simulink model "turbo_controller"  (R2025a)
settings: Solver=FixedStepAuto  StartTime=0.0  StopTime=inf  FixedStep=0.001  RelTol=1e-3
PostLoadFcn:
  | % 自动定位同目录CubeMX文件；不需要外部初始化脚本。
  | codertarget.data.setParameterValue('turbo_controller','STM32CubeMX.ProjectFile',fullfile(fileparts(get_param('turbo_controller','FileName')),'turbo_f407.ioc'));
InitFcn:
  | % 中文说明：按原控制器字段与类型创建三组接口总线；控制参数已内嵌。
  | tc_names=["EValve_Cycle" "EValve_Open" "Eblast_Cycle" "Eblast_Open" "Motor_Cycle" "Motor_Open" "EValve_Enable" "Eblast_Enable" "Motor_Enable" "SWO_Firework" "SWO_BleedAir" "EngineState" "Flag_ECUReset_Clear" "Flag_ECUReset_Save" "Flag_Reset_Enable" "Accelerator" "Nc_dem" "Nc"]; tc_types=["uint16" "uint16" "uint16" "uint16" "uint16" "uint16" "uint8" "uint8" "uint8" "uint8" "uint8" "uint8" "uint8" "uint8" "uint8" "single" "single" "single"];
  | for tc_k=1:numel(tc_names)
  |  tc_e(tc_k)=Simulink.BusElement; tc_e(tc_k).Name=char(tc_names(tc_k)); tc_e(tc_k).DataType=char(tc_types(tc_k));
  | end
  | EngineControl_Out=Simulink.Bus; EngineControl_Out.DataScope='Exported'; EngineControl_Out.Elements=tc_e;
  | clear tc_e tc_names tc_types tc_k
  | tc_names=["savedata1" "savedata2" "savedata3" "savedata4" "savedata5" "savedata6" "savedata7" "savedata8" "savedata9" "savedata10" "savedata11" "savedata12" "savedata13" "savedata14" "savedata15" "savedata16" "savedata17" "savedata18" "savedata19" "savedata20" "savedata21" "savedata22" "savedata23" "savedata24" "savedata25"]; tc_types=["single" "single" "single" "single" "single" "single" "single" "single" "single" "single" "single" "single" "single" "single" "single" "single" "single" "single" "single" "single" "single" "single" "single" "single" "single"];
  | for tc_k=1:numel(tc_names)
  |  tc_e(tc_k)=Simulink.BusElement; tc_e(tc_k).Name=char(tc_names(tc_k)); tc_e(tc_k).DataType=char(tc_types(tc_k));
  | end
  | SaveData_Out=Simulink.Bus; SaveData_Out.DataScope='Exported'; SaveData_Out.Elements=tc_e;
  | clear tc_e tc_names tc_types tc_k
  | tc_names=["senddata1" "senddata2" "senddata3" "senddata4" "senddata5" "senddata6" "senddata7" "senddata8" "senddata9" "senddata10" "senddata11" "senddata12" "senddata13" "senddata14" "senddata15" "senddata16" "senddata17" "senddata18" "senddata19" "senddata20" "senddata21" "senddata22" "senddata23" "senddata24" "senddata25" "senddata26" "senddata27" "senddata28" "senddata29"]; tc_types=["uint8" "uint8" "uint8" "uint8" "uint8" "uint8" "uint8" "uint8" "uint8" "uint8" "uint8" "uint8" "uint8" "uint8" "uint8" "uint8" "uint8" "uint8" "uint8" "uint8" "uint8" "uint8" "uint8" "uint8" "uint8" "uint8" "uint8" "uint8" "uint8"];
  | for tc_k=1:numel(tc_names)
  |  tc_e(tc_k)=Simulink.BusElement; tc_e(tc_k).Name=char(tc_names(tc_k)); tc_e(tc_k).DataType=char(tc_types(tc_k));
  | end
  | SendData_Out=Simulink.Bus; SendData_Out.DataScope='Exported'; SendData_Out.Elements=tc_e;
  | clear tc_e tc_names tc_types tc_k
  | 
  | % 以下为接口中文说明；只设置描述，不改变数值或数据类型。
  | EngineControl_Out.Description='执行控制输出（阀、电机、点火、状态及复位请求）';
  | tc_cn=["EValve_Cycle（主油阀周期计数（每计数2毫秒））" "EValve_Open（主油阀开通计数（每计数2毫秒））" "Eblast_Cycle（副油阀周期计数（每计数2毫秒））" "Eblast_Open（副油阀开通计数（每计数2毫秒））" "Motor_Cycle（起动电机周期计数）" "Motor_Open（起动电机开通计数）" "EValve_Enable（主油阀驱动使能）" "Eblast_Enable（副油阀驱动使能）" "Motor_Enable（起动电机使能）" "SWO_Firework（点火器使能（1开））" "SWO_BleedAir（引气阀使能（1开））" "EngineState（发动机状态）" "Flag_ECUReset_Clear（清除复位恢复状态请求）" "Flag_ECUReset_Save（保存复位恢复数据请求）" "Flag_Reset_Enable（处理器软件复位请求）" "Accelerator（油门／油泵给定控制量）" "Nc_dem（控制目标转速）" "Nc（发动机反馈转速（转每分））"];
  | tc_elements=EngineControl_Out.Elements;
  | for tc_k=1:numel(tc_cn)
  |  tc_elements(tc_k).Description=char(tc_cn(tc_k));
  | end
  | EngineControl_Out.Elements=tc_elements;
  | clear tc_cn tc_elements tc_k
  | SaveData_Out.Description='25项运行记录；字段含义按当前模型数据来源解释';
  | tc_cn=["savedata1（指令回显记录）" "savedata2（入口总温记录（℃））" "savedata3（电源电压记录）" "savedata4（排气温度记录（℃））" "savedata5（标定燃油压力记录）" "savedata6（副油阀占空比记录（％））" "savedata7（主油阀占空比记录（％））" "savedata8（温度修正转速记录）" "savedata9（开关输出及反馈位域）" "savedata10（物理转速记录）" "savedata11（油泵目标给定原始值）" "savedata12（起动电机占空比记录（％））" "savedata13（发动机状态码记录）" "savedata14（故障告警位域记录）" "savedata15（模型记录帧序号）" "savedata16（处理器温度记录（℃））" "savedata17（装订转速记录（沿用旧电源字段名））" "savedata18（导航高度记录）" "savedata19（飞行空速记录）" "savedata20（主阀旧记录位（恒零保留））" "savedata21（第21项保留记录（恒零））" "savedata22（保留记录项22）" "savedata23（保留记录项23）" "savedata24（保留记录项24）" "savedata25（保留记录项25）"];
  | tc_elements=SaveData_Out.Elements;
  | for tc_k=1:numel(tc_cn)
  |  tc_elements(tc_k).Description=char(tc_cn(tc_k));
  | end
  | SaveData_Out.Elements=tc_elements;
  | clear tc_cn tc_elements tc_k
  | SendData_Out.Description='29字段回传及外设命令接口；板端上位机帧只取第3至27字段';
  | tc_cn=["senddata1（回传发送允许标志（不直接上线路））" "senddata2（回传载荷长度25字节）" "senddata3（回传指令回显字节）" "senddata4（总温编码字节（℃＋80））" "senddata5（电源电压编码字节）" "senddata6（排温编码高字节）" "senddata7（排温编码低字节）" "senddata8（燃油压力编码高字节）" "senddata9（燃油压力编码低字节）" "senddata10（副油阀占空比字节（％））" "senddata11（主油阀占空比字节（％））" "senddata12（修正转速编码高字节）" "senddata13（修正转速编码低字节）" "senddata14（驱动及反馈状态位域）" "senddata15（物理转速编码高字节）" "senddata16（物理转速编码低字节）" "senddata17（油泵目标给定高字节（串口二使用））" "senddata18（油泵目标给定低字节（串口二使用））" "senddata19（起动电机占空比命令（串口一使用））" "senddata20（发动机状态码字节）" "senddata21（故障告警位域字节）" "senddata22（帧序号占位（板端另行填写））" "senddata23（处理器温度编码（℃＋50））" "senddata24（控制目标转速编码高字节）" "senddata25（控制目标转速编码低字节）" "senddata26（占位字节（板端改填实测泵速高字节））" "senddata27（占位字节（板端改填实测泵速低字节））" "senddata28（装订转速高字节（本板未发送））" "senddata29（装订转速低字节（本板未发送））"];
  | tc_elements=SendData_Out.Elements;
  | for tc_k=1:numel(tc_cn)
  |  tc_elements(tc_k).Description=char(tc_cn(tc_k));
  | end
  | SendData_Out.Elements=tc_elements;
  | clear tc_cn tc_elements tc_k
  | 
  | 
  | % FRAM模块化事务：接口类型和上电初始状态，随模型保存，无外部初始化文件。
  | clear FM_elements
  | FM_elements(1)=Simulink.BusElement;FM_elements(1).Name='phase';FM_elements(1).DataType='uint8';FM_elements(1).Dimensions=[1 1];FM_elements(1).Description='phase（当前事务阶段）';
  | FM_elements(2)=Simulink.BusElement;FM_elements(2).Name='a';FM_elements(2).DataType='uint8';FM_elements(2).Dimensions=[64 1];FM_elements(2).Description='a（启动时缓存的首区64字节）';
  | FM_elements(3)=Simulink.BusElement;FM_elements(3).Name='active';FM_elements(3).DataType='uint16';FM_elements(3).Dimensions=[1 1];FM_elements(3).Description='active（当前有效记录区地址）';
  | FM_elements(4)=Simulink.BusElement;FM_elements(4).Name='generation';FM_elements(4).DataType='uint32';FM_elements(4).Dimensions=[1 1];FM_elements(4).Description='generation（当前有效记录代号）';
  | FM_elements(5)=Simulink.BusElement;FM_elements(5).Name='record';FM_elements(5).DataType='uint8';FM_elements(5).Dimensions=[64 1];FM_elements(5).Description='record（本次冻结的待写记录）';
  | FM_elements(6)=Simulink.BusElement;FM_elements(6).Name='addr';FM_elements(6).DataType='uint16';FM_elements(6).Dimensions=[1 1];FM_elements(6).Description='addr（本次备用写入地址）';
  | FM_elements(7)=Simulink.BusElement;FM_elements(7).Name='lastSave';FM_elements(7).DataType='single';FM_elements(7).Dimensions=[1 1];FM_elements(7).Description='lastSave（上次开始保存的秒数）';
  | FM_elements(8)=Simulink.BusElement;FM_elements(8).Name='lastState';FM_elements(8).DataType='uint8';FM_elements(8).Dimensions=[1 1];FM_elements(8).Description='lastState（上次保存时的发动机状态）';
  | FM_elements(9)=Simulink.BusElement;FM_elements(9).Name='boot';FM_elements(9).DataType='boolean';FM_elements(9).Dimensions=[1 1];FM_elements(9).Description='boot（启动记录是否允许恢复）';
  | FM_elements(10)=Simulink.BusElement;FM_elements(10).Name='consumed';FM_elements(10).DataType='boolean';FM_elements(10).Dimensions=[1 1];FM_elements(10).Description='consumed（本次启动恢复通知是否已发送）';
  | FM_elements(11)=Simulink.BusElement;FM_elements(11).Name='payload';FM_elements(11).DataType='uint8';FM_elements(11).Dimensions=[20 1];FM_elements(11).Description='payload（当前20字节恢复内容）';
  | ... (+35 lines)
model workspace (MAT data in the model file):
  CRC16_Table_Reference = [0 4129 8258 12387 16516 20645 24774 28903 33032 37161 41290 45419 ... (256 elements, 256x1)]
  PE_Kaer = [0.15402 0.15402 0.12264 0.10076 0.09481 0.07601 0.07111 0.0569 0.05198 0.04926 0.05308 0.04325 ... (13 elements, 1x13)]
  PE_Nr = [21.2982 61.4260372 67.7475458 72.7394382 76.845934 80.6988798 83.8449282 86.6491912 88.9382406 89.178606 91.1938214 93.4068058 ... (13 elements, 1x13)]
  PE_Pump_Translate = 33.5999984741
  PE_RotaSpeed_Translate = 860
  PE_Taer = [0.4939154 0.4939154 0.40780982 0.34066978 0.31622756 0.30405716 0.34300244 0.26785022 0.37393554 0.23914836 0.44563948 0.31044662 ... (13 elements, 1x13)]
  PF_ACCFULLRANGE = 3360
  PF_Flag_ECUReset = 0
  PF_Flag_rx_suc = 1
  PF_Gear_Info = [40000; 45000; 50000; 55000; 57000; 59000; 60000; 61000; 61000; 61000; 61000; 61000]
  PF_K_TiaoJie = 1
  PF_Kpu = 10
  PF_MySet_Rxdata = [0 0 0 0 0 0 0 0 0 0 0 0 ... (50 elements, 50x1)]
  PF_MyUsart1_Rxdata = [0 0 0 0 0 0 0 0 0 0 0 0 ... (50 elements, 50x1)]
  PF_MyUsart2_Rxdata = [0 0 0 0 0 0 0 0 0 0 0 0 ... (50 elements, 50x1)]
  PF_Reset_Information = [0 0 0 0 0 0 0 0 0 0 0 0 ... (20 elements, 20x1)]
  PF_Sensor_X1_T4 = [0 4095]
  PF_Sensor_X2_T4 = [0 1.66666698456]
  PF_Sensor_X3_T4 = [0 504 999 1497 2010 2529 3051 3568 4076 4571 4959]
  PF_Sensor_X_P2 = [0.5 3]
  PF_Sensor_X_Poil = [0.5 3]
  PF_Sensor_X_T1t = [-50 300]
  PF_Sensor_X_Vpower = [0 3]
  PF_Sensor_X_Vpump = [0 3]
  PF_Sensor_Y1_T4 = [0 3]
  PF_Sensor_Y2_T4 = [0 5000]
  PF_Sensor_Y3_T4 = [0 100 200 300 400 500 600 700 800 900 980]
  PF_Sensor_Y_P2 = [0 1000]
  PF_Sensor_Y_Poil = [0 1000]
  PF_Sensor_Y_T1t = [-50 300]
  PF_Sensor_Y_Vpower = [0 33]
  PF_Sensor_Y_Vpump = [0 33]
  PG_CtrlMode_CloseLoop : mpt.Parameter (value not decoded)
  PG_CtrlMode_ManualAcc : mpt.Parameter (value not decoded)
  PG_CtrlMode_Origin : mpt.Parameter (value not decoded)
  PG_CtrlMode_Start : mpt.Parameter (value not decoded)
  PG_CtrlMode_Stop : mpt.Parameter (value not decoded)
  PG_ES_Clp : mpt.Parameter (value not decoded)
  PG_ES_EngStart : mpt.Parameter (value not decoded)
  PG_ES_Manual : mpt.Parameter (value not decoded)
  PG_ES_Origin : mpt.Parameter (value not decoded)
  PG_ES_Stop : mpt.Parameter (value not decoded)
  PG_Instr_BleedAirSet : mpt.Parameter (value not decoded)
  PG_Instr_CloseLoop : mpt.Parameter (value not decoded)
  PG_Instr_ECUReSet : mpt.Parameter (value not decoded)
  PG_Instr_EValveSet : mpt.Parameter (value not decoded)
  PG_Instr_EblastSet : mpt.Parameter (value not decoded)
  PG_Instr_Erase : mpt.Parameter (value not decoded)
  PG_Instr_FireWorkSet : mpt.Parameter (value not decoded)
  PG_Instr_ManualPlus : mpt.Parameter (value not decoded)
  PG_Instr_ManualrReduce : mpt.Parameter (value not decoded)
  PG_Instr_MotorSet : mpt.Parameter (value not decoded)
  PG_Instr_OilSet : mpt.Parameter (value not decoded)
  PG_Instr_SelfCheck : mpt.Parameter (value not decoded)
  PG_Instr_Start : mpt.Parameter (value not decoded)
  PG_Instr_Stop : mpt.Parameter (value not decoded)
  PG_Instr_StopZero : Simulink.Parameter (value not decoded)
  PG_Location_Air : Simulink.Parameter (value not decoded)
  PG_Location_Gnd : Simulink.Parameter (value not decoded)
  PG_ServoCtrlMode_CloseLoop : Simulink.Parameter (value not decoded)
  PG_ServoCtrlMode_CloseLoopMax : Simulink.Parameter (value not decoded)
  PG_ServoCtrlMode_CloseLoopMin : Simulink.Parameter (value not decoded)
  PG_ServoCtrlMode_ManualAcc : Simulink.Parameter (value not decoded)
  PG_ServoCtrlMode_ManualAccMax : Simulink.Parameter (value not decoded)
  PG_ServoCtrlMode_ManualAccMin : Simulink.Parameter (value not decoded)
  PG_SpeedDot_Permit : Simulink.Parameter (value not decoded)
  PL_EngineModel_Actuator = [0 10 100]
  PL_EngineModel_EngineStar_Press_P2 = [1013 1098.4 1099.144828 1099.931034 1103.613793 1162.662069 1143.793103 1131.006897 1123.186207 1117.6 1114 1111.806897 ... (127 elements, 1x127)]
  PL_EngineModel_EngineStar_RotaSpeed = [200 2000 9584 9660 10220 10240 10260 10288 10308 10368 10380 10408 ... (127 elements, 1x127)]
  PL_EngineModel_EngineStar_Temp_Exhaust = [128 129 129.1 130 131 131.1 132 133 134 134.1 135 135.1 ... (127 elements, 1x127)]
  PL_EngineModel_EngineStar_Time = [0.05 0.1 0.15 0.2 0.25 0.3 0.35 0.4 0.45 0.5 0.55 0.6 ... (127 elements, 1x127)]
  PL_EngineModel_IdleAbove_Nr = [0 21.2982 61.4260372 67.7475458 72.7394382 76.845934 80.6988798 83.8449282 86.6491912 88.9382406 89.178606 91.1938214 ... (14 elements, 1x14)]
  PL_EngineModel_IdleAbove_P2r = [0.986923266716 1.57907722675 1.81593881076 1.99358499877 2.23044658278 2.43770046879 2.65482358747 2.84233900814 3.03972366149 3.18776215149 3.25684678016 3.3950160375 ... (14 elements, 1x14)]
  PL_EngineModel_IdleAbove_Tempr = [0.0536001429337 1.07200285867 1.63301768805 1.63659103091 1.66875111667 1.72592460247 1.77595140254 1.86171163123 1.95461854565 2.03323208862 2.03323208862 2.13685903162 ... (14 elements, 1x14)]
  PL_EngineModel_IdleAbove_Ter = [0.42434128 0.42434128 0.42434128 0.30669408 0.23570008 0.22150128 0.1997974 0.23803274 0.16115638 0.24279948 0.13600422 0.31308354 ... (14 elements, 1x14)]
  PL_EngineModel_IdleAbove_Wfr = [0 10.142 23.8337 27.8905 31.9473 36.0041 40.0609 44.1177 48.1745 52.2313 52.7384 56.7952 ... (14 elements, 1x14)]
  PL_EngineModel_Press_P2 = [400 400 400 400 400 400 400 400 400 400]
  PL_EngineModel_Rotaspeed = [0 20000 96400]
  PL_EngineModel_Temp_Exhaust = [500 500 500 500 500 500 500 500 500 500]
  PL_Kaer = [0.1 0.1 0.1 0.1 0.1 0.1]
  PL_Nr = [50 60 70 80 90 100]
  PL_Taer = [0.1 0.1 0.1 0.1 0.1 0.1]
  Sig : Simulink.Signal (value not decoded)
  Ts_ms : Simulink.Parameter (value not decoded)
  false : Simulink.Parameter (value not decoded)
  true : Simulink.Parameter (value not decoded)
symbols that are objects in the model workspace (value not decoded): PG_CtrlMode_CloseLoop, PG_CtrlMode_ManualAcc, PG_CtrlMode_Origin, PG_CtrlMode_Start, PG_CtrlMode_Stop, PG_ES_Clp, PG_ES_EngStart, PG_ES_Manual, PG_ES_Origin, PG_ES_Stop, PG_Instr_BleedAirSet, PG_Instr_CloseLoop, PG_Instr_EblastSet, PG_Instr_ECUReSet, PG_Instr_Erase, PG_Instr_EValveSet, PG_Instr_FireWorkSet, PG_Instr_ManualPlus, PG_Instr_ManualrReduce, PG_Instr_MotorSet, PG_Instr_OilSet, PG_Instr_SelfCheck, PG_Instr_Start, PG_Instr_Stop, PG_Instr_StopZero, PG_ServoCtrlMode_CloseLoop, PG_ServoCtrlMode_CloseLoopMax, PG_ServoCtrlMode_CloseLoopMin, PG_ServoCtrlMode_ManualAcc, PG_ServoCtrlMode_ManualAccMax, PG_ServoCtrlMode_ManualAccMin, Ts_ms
libraries: simulink x97, stm32blockslib x10, stm32f4xxblockslib x8
(part 24 of 26)

== system turbo_controller/BoardInput_输入换算与协议解析/In03_Pump（油泵回包预留校验）/Receive（逐字节组帧与保持有效结果）_353/Step03_收齐且校验通过才接受/Verify（完整帧校验）_344/CRC16（循环冗余校验）_328/TableStep（查表更新本字节校验） ==
  note: CRC16的一个字节怎样查表更新
      |
      | 父级已经把当前数据字节异或进旧CRC的高8位，形成Merged。本模块把这个16位数拆成“用哪项表”和
      | “保留哪些移位结果”两部分。
      |
      | 先取高8位：索引=floor(Merged/256)，范围0～255。用它到CRC16_Table_Reference查表；模型Select
      | or按零基索引取值，写成MATLAB数组下标时要用索引+1。
      | 另一条支路把Merged左移一个字节，即乘256，然后只保留低16位：移位值=bitand(uint32(Merged)×25
      | 6,65535)。
      |
      | 最后将表值与移位值按位异或：
      | 新CRC=bitxor(表值,移位值)。
      |
      | 例如Merged=十六进制1234，高8位12用于选表项，左移并截16位后为3400，再与表项异或。宽类型uint
      | 32是为了中间计算不先溢出，并不表示输出CRC变成32位。结果回到父级，继续处理下一个数据字节。
  note: 【中文学习说明：一次查表更新一个字节】
      | 一、输入已经是“旧CRC XOR (当前字节×256)”。
      | 输入是16位无符号整数，记作Merged（合并值）。
      |
      | 二、上路得到查表下标。
      | 合并值÷256后向下取整，取得高八位，范围0～255。
      | 这等价于参考程序中的“旧CRC高字节 XOR 当前字节”。
      | Lookup（按下标取表项）采用Zero-based（从0编号），
      | 所以0就取表的第一项，255取最后一项，不能再加1。
      |
      | 三、下路准备左移结果。
      | 先转uint32（32位无符号数），再乘256左移8位，
      | 与65535作按位AND，只保留低16位，最后转回uint16。
      | 先加宽再移位，是为了避免整数饱和破坏结果。
      | 当前字节已经在高8位，左移后移出16位范围，
      | 因此截断后与“旧CRC左移8位”的结果相同。
      |
      | 四、两路按位XOR（异或），输出更新后的16位CRC。
      | 异或的意思：两个二进制位相同得0，不同得1。
      | 本页不需要循环和记忆，输入一到就能按组合逻辑计算；
      | 跨字节的累计和每帧初值由父级CRC16模块负责。
      |
      | 五、CRC16Table（查表数据）是256项整数常量。
      | 表内容逐项复制自参考工程USER/crc.c，
      | 与NRIST_lib/NRIST_calculate.c中的表一致。
      | Selector（按下标选取）直接取一项，不做曲线插值。
      | 表中数值不是需要现场调节的控制参数。
  Merged（旧校验值与当前字节异或后的数） : Inport  OutDataTypeStr=uint16
  CRC16Table（参考工程原始二百五十六项表） : Constant  Value=CRC16_Table_Reference  OutDataTypeStr=uint16
  Divisor（高字节换算除数） : Constant  Value=256  OutDataTypeStr=double
  Exact（转双精度做精确除法） : DataTypeConversion  OutDataTypeStr=double  SaturateOnIntegerOverflow=off  RndMeth=Floor
  HighByte（除二百五十六取高字节） : Product  Inputs=*/  OutDataTypeStr=double
  Index（向下取整得到零至二百五十五） : DataTypeConversion  OutDataTypeStr=uint32  RndMeth=Floor
  LeftByte（左移一个字节） : Product  Inputs=**  OutDataTypeStr=uint32  SaturateOnIntegerOverflow=on
  Lookup（按零基索引读取校验表） : Selector  IndexMode=Zero-based  InputPortWidth=256  IndexOptions=Index vector (port)  Indices=1  OutputSizes=1
  Mask16（保留低十六位） : Constant  Value=65535  OutDataTypeStr=uint32
  Shift16（移位结果转十六位） : DataTypeConversion  OutDataTypeStr=uint16  SaturateOnIntegerOverflow=off  RndMeth=Floor
  ShiftBase（一个字节的移位系数） : Constant  Value=256  OutDataTypeStr=uint32
  Update（查表值与移位结果异或） : simulink/Logic and Bit Operations/Bitwise Operator  logicop=XOR  UseBitMask=off  NumInputPorts=2  BitMask=bin2dec('11011001')  BitMaskRealWorld=Stored Integer
      settings: LibrarySourceBlock=|
      | hdlsllib/Logic and Bit
      | Operations/Bitwise
      | Operator
  Wide（转三十二位防止移位溢出） : DataTypeConversion  OutDataTypeStr=uint32  SaturateOnIntegerOverflow=off  RndMeth=Floor
  Wrap16（截取左移后的低十六位） : simulink/Logic and Bit Operations/Bitwise Operator  logicop=AND  UseBitMask=off  NumInputPorts=2  BitMask=bin2dec('11011001')  BitMaskRealWorld=Stored Integer
      settings: LibrarySourceBlock=|
      | hdlsllib/Logic and Bit
      | Operations/Bitwise
      | Operator
  CRC（本字节处理后的校验值） : Outport
  wires:
  Merged（旧校验值与当前字节异或后的数）/1 -> Wide（转三十二位防止移位溢出）/1, Exact（转双精度做精确除法）/1
  Wide（转三十二位防止移位溢出）/1 -> LeftByte（左移一个字节）/1
  ShiftBase（一个字节的移位系数）/1 -> LeftByte（左移一个字节）/2
  LeftByte（左移一个字节）/1 -> Wrap16（截取左移后的低十六位）/1
  Mask16（保留低十六位）/1 -> Wrap16（截取左移后的低十六位）/2
  Wrap16（截取左移后的低十六位）/1 -> Shift16（移位结果转十六位）/1
  Exact（转双精度做精确除法）/1 -> HighByte（除二百五十六取高字节）/1
  Divisor（高字节换算除数）/1 -> HighByte（除二百五十六取高字节）/2
  HighByte（除二百五十六取高字节）/1 -> Index（向下取整得到零至二百五十五）/1
  CRC16Table（参考工程原始二百五十六项表）/1 -> Lookup（按零基索引读取校验表）/1
  Index（向下取整得到零至二百五十五）/1 -> Lookup（按零基索引读取校验表）/2
  Lookup（按零基索引读取校验表）/1 -> Update（查表值与移位结果异或）/1
  Shift16（移位结果转十六位）/1 -> Update（查表值与移位结果异或）/2
  Update（查表值与移位结果异或）/1 -> CRC（本字节处理后的校验值）/1

== system turbo_controller/BoardOutput_串口封装与阀门时序/Out01_Pump（泵反馈解析与滤波）/Receive（逐字节组帧与保持有效结果）_680/Step03_收齐且校验通过才接受/Verify（完整帧校验）_662/CRC16（循环冗余校验）_646/TableStep（查表更新本字节校验） ==
  note: CRC16的一个字节怎样查表更新
      |
      | 父级已经把当前数据字节异或进旧CRC的高8位，形成Merged。本模块把这个16位数拆成“用哪项表”和
      | “保留哪些移位结果”两部分。
      |
      | 先取高8位：索引=floor(Merged/256)，范围0～255。用它到CRC16_Table_Reference查表；模型Select
      | or按零基索引取值，写成MATLAB数组下标时要用索引+1。
      | 另一条支路把Merged左移一个字节，即乘256，然后只保留低16位：移位值=bitand(uint32(Merged)×25
      | 6,65535)。
      |
      | 最后将表值与移位值按位异或：
      | 新CRC=bitxor(表值,移位值)。
      |
      | 例如Merged=十六进制1234，高8位12用于选表项，左移并截16位后为3400，再与表项异或。宽类型uint
      | 32是为了中间计算不先溢出，并不表示输出CRC变成32位。结果回到父级，继续处理下一个数据字节。
  note: 【中文学习说明：一次查表更新一个字节】
      | 一、输入已经是“旧CRC XOR (当前字节×256)”。
      | 输入是16位无符号整数，记作Merged（合并值）。
      |
      | 二、上路得到查表下标。
      | 合并值÷256后向下取整，取得高八位，范围0～255。
      | 这等价于参考程序中的“旧CRC高字节 XOR 当前字节”。
      | Lookup（按下标取表项）采用Zero-based（从0编号），
      | 所以0就取表的第一项，255取最后一项，不能再加1。
      |
      | 三、下路准备左移结果。
      | 先转uint32（32位无符号数），再乘256左移8位，
      | 与65535作按位AND，只保留低16位，最后转回uint16。
      | 先加宽再移位，是为了避免整数饱和破坏结果。
      | 当前字节已经在高8位，左移后移出16位范围，
      | 因此截断后与“旧CRC左移8位”的结果相同。
      |
      | 四、两路按位XOR（异或），输出更新后的16位CRC。
      | 异或的意思：两个二进制位相同得0，不同得1。
      | 本页不需要循环和记忆，输入一到就能按组合逻辑计算；
      | 跨字节的累计和每帧初值由父级CRC16模块负责。
      |
      | 五、CRC16Table（查表数据）是256项整数常量。
      | 表内容逐项复制自参考工程USER/crc.c，
      | 与NRIST_lib/NRIST_calculate.c中的表一致。
      | Selector（按下标选取）直接取一项，不做曲线插值。
      | 表中数值不是需要现场调节的控制参数。
  Merged（旧校验值与当前字节异或后的数） : Inport  OutDataTypeStr=uint16
  CRC16Table（参考工程原始二百五十六项表） : Constant  Value=CRC16_Table_Reference  OutDataTypeStr=uint16
  Divisor（高字节换算除数） : Constant  Value=256  OutDataTypeStr=double
  Exact（转双精度做精确除法） : DataTypeConversion  OutDataTypeStr=double  SaturateOnIntegerOverflow=off  RndMeth=Floor
  HighByte（除二百五十六取高字节） : Product  Inputs=*/  OutDataTypeStr=double
  Index（向下取整得到零至二百五十五） : DataTypeConversion  OutDataTypeStr=uint32  RndMeth=Floor
  LeftByte（左移一个字节） : Product  Inputs=**  OutDataTypeStr=uint32  SaturateOnIntegerOverflow=on
  Lookup（按零基索引读取校验表） : Selector  IndexMode=Zero-based  InputPortWidth=256  IndexOptions=Index vector (port)  Indices=1  OutputSizes=1
  Mask16（保留低十六位） : Constant  Value=65535  OutDataTypeStr=uint32
  Shift16（移位结果转十六位） : DataTypeConversion  OutDataTypeStr=uint16  SaturateOnIntegerOverflow=off  RndMeth=Floor
  ShiftBase（一个字节的移位系数） : Constant  Value=256  OutDataTypeStr=uint32
  Update（查表值与移位结果异或） : simulink/Logic and Bit Operations/Bitwise Operator  logicop=XOR  UseBitMask=off  NumInputPorts=2  BitMask=bin2dec('11011001')  BitMaskRealWorld=Stored Integer
      settings: LibrarySourceBlock=|
      | hdlsllib/Logic and Bit
      | Operations/Bitwise
      | Operator
  Wide（转三十二位防止移位溢出） : DataTypeConversion  OutDataTypeStr=uint32  SaturateOnIntegerOverflow=off  RndMeth=Floor
  Wrap16（截取左移后的低十六位） : simulink/Logic and Bit Operations/Bitwise Operator  logicop=AND  UseBitMask=off  NumInputPorts=2  BitMask=bin2dec('11011001')  BitMaskRealWorld=Stored Integer
      settings: LibrarySourceBlock=|
      | hdlsllib/Logic and Bit
      | Operations/Bitwise
      | Operator
  CRC（本字节处理后的校验值） : Outport
  wires:
  Merged（旧校验值与当前字节异或后的数）/1 -> Wide（转三十二位防止移位溢出）/1, Exact（转双精度做精确除法）/1
  Wide（转三十二位防止移位溢出）/1 -> LeftByte（左移一个字节）/1
  ShiftBase（一个字节的移位系数）/1 -> LeftByte（左移一个字节）/2
  LeftByte（左移一个字节）/1 -> Wrap16（截取左移后的低十六位）/1
  Mask16（保留低十六位）/1 -> Wrap16（截取左移后的低十六位）/2
  Wrap16（截取左移后的低十六位）/1 -> Shift16（移位结果转十六位）/1
  Exact（转双精度做精确除法）/1 -> HighByte（除二百五十六取高字节）/1
  Divisor（高字节换算除数）/1 -> HighByte（除二百五十六取高字节）/2
  HighByte（除二百五十六取高字节）/1 -> Index（向下取整得到零至二百五十五）/1
  CRC16Table（参考工程原始二百五十六项表）/1 -> Lookup（按零基索引读取校验表）/1
  Index（向下取整得到零至二百五十五）/1 -> Lookup（按零基索引读取校验表）/2
  Lookup（按零基索引读取校验表）/1 -> Update（查表值与移位结果异或）/1
  Shift16（移位结果转十六位）/1 -> Update（查表值与移位结果异或）/2
  Update（查表值与移位结果异或）/1 -> CRC（本字节处理后的校验值）/1

== stateflow chart turbo_controller/MAM/Timmer_ms1 ==
  note: 确认越限是否持续达到指定时间
      |
      | 输入越限条件成立时累计次数；不成立时按图内复位分支清除本次确认。到Time_ms/Ts_ms对应的门限
      | 后，输出持续越限标志。
      |
      | 父级给定约2000 ms，Ts_ms=20 ms，相当于约100次连续调用。温度或转速只超过一拍后恢复，不会累
      | 计成连续2 s。该定时只用于告警确认，不改变测量值，也不对排温或转速再次滤波。
  (default) -> (junction 26)
    settings: description=无附加条件的迁移路径，执行次序1；沿本图当前连接推进。
  (junction 26) -> (junction 3) [order 1] : [true/*真值*/ == In/*输入*/]
    settings: description=本路径的判据/动作：[true == In]。执行次序1；条件成立才执行本箭头动作。
  (junction 3) -> (junction 5) [order 1] : [Cnt/*计数器*/ >= uint32/*三十二位无符号整数*/(100000)]
    settings: description=本路径的判据/动作：[Cnt >= uint32(100000)]。执行次序1；条件成立才执行本箭头动作。
  (junction 26) -> (junction 43) [order 2] : {Cnt/*计数器*/ = 0;Out/*输出*/ = false/*假值*/;}
    settings: description=本路径的判据/动作：{Cnt = 0;Out = false;}。执行次序2；条件成立才执行本箭头动作。
  (junction 3) -> (junction 10) [order 2] : {Cnt/*计数器*/++;}
    settings: description=本路径的判据/动作：{Cnt++;}。执行次序2；条件成立才执行本箭头动作。
  (junction 5) -> (junction 12) : {Cnt/*计数器*/ = 100000;}
    settings: description=本路径的判据/动作：{Cnt = 100000;}。执行次序1；条件成立才执行本箭头动作。
  (junction 12) -> (junction 10)
    settings: description=无附加条件的迁移路径，执行次序1；沿本图当前连接推进。
  (junction 10) -> (junction 30)
    settings: description=无附加条件的迁移路径，执行次序1；沿本图当前连接推进。
  (junction 30) -> (junction 33) [order 1] : [Cnt/*计数器*/ >uint32/*三十二位无符号整数*/(Time_ms/*时间毫秒*//Ts_ms/*采样周期毫秒*/)]
    settings: description=本路径的判据/动作：[Cnt >uint32(Time_ms/Ts_ms)]。执行次序1；条件成立才执行本箭头动作。
  (junction 30) -> (junction 37) [order 2] : {Out/*输出*/ = false/*假值*/;}
    settings: description=本路径的判据/动作：{Out = false;}。执行次序2；条件成立才执行本箭头动作。
  (junction 33) -> (junction 36) : {Out/*输出*/ = true/*真值*/;}
    settings: description=本路径的判据/动作：{Out = true;}。执行次序1；条件成立才执行本箭头动作。
  (junction 36) -> (junction 37)
    settings: description=无附加条件的迁移路径，执行次序1；沿本图当前连接推进。
  (junction 37) -> (junction 55)
    settings: description=无附加条件的迁移路径，执行次序1；沿本图当前连接推进。
  (junction 55) -> (junction 43)
    settings: description=无附加条件的迁移路径，执行次序1；沿本图当前连接推进。
  (junction 43) -> (junction 71)
    settings: description=无附加条件的迁移路径，执行次序1；沿本图当前连接推进。
  data: Cnt local uint32 =0; Out output boolean =0; In input boolean; Time_ms input single; Ts_ms parameter single

== stateflow chart turbo_controller/ESM/StateTransition/StateTranslation ==
  note: 保存五种发动机模式，并按允许条件切换
      |
      | 初始为Origin，对外编号0。收到相应转换标志后，可以进入普通Start=1、闭环Clp=2或手动Manual=3
      | ；运行过程中停车请求进入Stop=4，停车完成并满足转速条件再回Origin。
      |
      | 每个状态的进入动作写EngineState，其他子系统读取这个编号决定运行哪套控制算法。转换的守卫条
      | 件来自Flags，起动是否完成则来自Start内部阶段结果。
      |
      | 本图是模式记忆：即便某个命令只出现一拍，已进入的模式也会保持到下一次合法转换。不能把命令编
      | 号、起动A～F阶段和这五种模式当作同一种“状态”。
  state Origin % 原位
    entry: % 进入时执行:
    EngineState = PG_ES_Origin; % 发动机状态 = 原位状态码;
  state Stop % 停车
    entry: % 进入时执行:
    EngineState = PG_ES_Stop; % 发动机状态 = 停车状态码;
  state Start % 地面起动
    entry: % 进入时执行:
    EngineState = PG_ES_EngStart; % 发动机状态 = 起动状态码;
  state IdleAndAbove % 慢车及以上
    entry: % 进入时执行:
    EngineState = PG_ES_Clp; % 发动机状态 = 闭环状态码;
  state Manual % 手动
    entry: % 进入时执行:
    EngineState = PG_ES_Manual; % 发动机状态 = 手动状态码;
  (default) -> Origin % 原位
    settings: description=无附加条件的迁移路径，执行次序1；沿本图当前连接推进。
  Origin % 原位 -> (junction 83) [order 2]
    settings: description=无附加条件的迁移路径，执行次序2；沿本图当前连接推进。
  (junction 83) -> (junction 120)
    settings: description=无附加条件的迁移路径，执行次序1；沿本图当前连接推进。
  Stop % 停车 -> Origin % 原位 : [true == Stop2Origin ... % 真 == 停车转原位
      | ]
    settings: description=本路径的判据/动作：[true == Stop2Origin ... % 真 == 停车转原位 ]。执行次序1；条件成立才执行本箭头动作。
  (junction 42) -> Stop % 停车
    settings: description=无附加条件的迁移路径，执行次序1；沿本图当前连接推进。
  (junction 41) -> (junction 42)
    settings: description=无附加条件的迁移路径，执行次序1；沿本图当前连接推进。
  Origin % 原位 -> Start % 地面起动 [order 1] : [true == Origin2Start ... % 真 == 原位转起动
      | ]
    settings: description=本路径的判据/动作：[true == Origin2Start ... % 真 == 原位转起动 ]。执行次序1；条件成立才执行本箭头动作。
  (junction 13) -> Stop % 停车
    settings: description=无附加条件的迁移路径，执行次序1；沿本图当前连接推进。
  (junction 12) -> (junction 13)
    settings: description=无附加条件的迁移路径，执行次序1；沿本图当前连接推进。
  Start % 地面起动 -> (junction 12) [order 2] : [true ==Start2Stop ... % 真 ==起动转停车
      | ]
    settings: description=本路径的判据/动作：[true ==Start2Stop ... % 真 ==起动转停车 ]。执行次序2；条件成立才执行本箭头动作。
  IdleAndAbove % 慢车及以上 -> (junction 13) [order 1] : [true == Clp2Stop ... % 真 == 闭环转停车
      | ]
    settings: description=本路径的判据/动作：[true == Clp2Stop ... % 真 == 闭环转停车 ]。执行次序1；条件成立才执行本箭头动作。
  Start % 地面起动 -> (junction 108) [order 1] : [true == Start2Clp ... % 真 == 起动转闭环
      | ]
    settings: description=本路径的判据/动作：[true == Start2Clp ... % 真 == 起动转闭环 ]。执行次序1；条件成立才执行本箭头动作。
  (junction 108) -> IdleAndAbove % 慢车及以上
    settings: description=无附加条件的迁移路径，执行次序1；沿本图当前连接推进。
  Start % 地面起动 -> Manual % 手动 [order 3] : [true == Start2Manual ... % 真 == 起动转手动
      | ]
    settings: description=本路径的判据/动作：[true == Start2Manual ... % 真 == 起动转手动 ]。执行次序3；条件成立才执行本箭头动作。
  (junction 120) -> (junction 106) [order 1] : [true == Origin2Clp ... % 真 == 原位转闭环
      | ]
    settings: description=本路径的判据/动作：[true == Origin2Clp ... % 真 == 原位转闭环 ]。执行次序1；条件成立才执行本箭头动作。
  (junction 106) -> IdleAndAbove % 慢车及以上
    settings: description=无附加条件的迁移路径，执行次序1；沿本图当前连接推进。
  (junction 120) -> (junction 90) [order 2] : [true == Origin2Manual ... % 真 == 原位转手动
      | ]
    settings: description=本路径的判据/动作：[true == Origin2Manual ... % 真 == 原位转手动 ]。执行次序2；条件成立才执行本箭头动作。
  Manual % 手动 -> (junction 106) [order 2] : [true == Manual2Clp ... % 真 == 手动转闭环
      | ]
    settings: description=本路径的判据/动作：[true == Manual2Clp ... % 真 == 手动转闭环 ]。执行次序2；条件成立才执行本箭头动作。
  IdleAndAbove % 慢车及以上 -> (junction 38) [order 2] : [true == Clp2Manual ... % 真 == 闭环转手动
      | ]
    settings: description=本路径的判据/动作：[true == Clp2Manual ... % 真 == 闭环转手动 ]。执行次序2；条件成立才执行本箭头动作。
  (junction 38) -> Manual % 手动
    settings: description=无附加条件的迁移路径，执行次序1；沿本图当前连接推进。
  Manual % 手动 -> (junction 41) [order 1] : [true == Manual2Stop ... % 真 == 手动转停车
      | ]
    settings: description=本路径的判据/动作：[true == Manual2Stop ... % 真 == 手动转停车 ]。执行次序1；条件成立才执行本箭头动作。
  (junction 90) -> Manual % 手动
    settings: description=无附加条件的迁移路径，执行次序1；沿本图当前连接推进。
  data: Origin2Start input boolean; Start2Clp input boolean; Clp2Stop input boolean; Stop2Origin input boolean; EngineState output uint8; PG_ES_Stop parameter; PG_ES_Origin parameter; PG_ES_EngStart parameter; PG_ES_Clp parameter; Manual2Clp input boolean; Manual2Stop input boolean; Start2Manual input boolean; Clp2Manual input boolean; PG_ES_Manual parameter; Start2Stop input boolean; Origin2Clp input boolean; Origin2Manual input boolean

== stateflow chart turbo_controller/FPM/Subsystem/Hold_2000ms ==
  note: 等待恢复条件持续约2 s后才置恢复控制标志
      |
      | Flag_ECUReset为真时累计次数，为假时立即清计数并令ResetControl为假。计数尚小于Time_ms/Ts_ms
      | 时输出假，达到门限后输出真。
      |
      | 当前Time_ms=2000、Ts_ms=20，对应100次调用。这样一次瞬时有效信号不会立即完成恢复确认。计数
      | 有10000封顶，避免持续有效时无限增长；输入撤销后需要重新累计。
  (default) -> (junction 26)
    settings: description=无附加条件的迁移路径，执行次序1；沿本图当前连接推进。
  (junction 26) -> (junction 3) [order 1] : [true/*真值*/ == Flag_ECUReset/*复位恢复标志*/]
    settings: description=本路径的判据/动作：[true == Flag_ECUReset]。执行次序1；条件成立才执行本箭头动作。
  (junction 3) -> (junction 5) [order 1] : [Cnt/*计数器*/ >= uint32/*三十二位无符号整数*/(10000)]
    settings: description=本路径的判据/动作：[Cnt >= uint32(10000)]。执行次序1；条件成立才执行本箭头动作。
  (junction 26) -> (junction 43) [order 2] : {Cnt/*计数器*/ = 0;
      | ResetControl/*复位控制*/ = false/*假值*/;}
    settings: description=本路径的判据/动作：{Cnt = 0; ResetControl = false;}。执行次序2；条件成立才执行本箭头动作。
  (junction 3) -> (junction 10) [order 2] : {Cnt/*计数器*/++;}
    settings: description=本路径的判据/动作：{Cnt++;}。执行次序2；条件成立才执行本箭头动作。
  (junction 5) -> (junction 12) : {Cnt/*计数器*/ = 10000;}
    settings: description=本路径的判据/动作：{Cnt = 10000;}。执行次序1；条件成立才执行本箭头动作。
  (junction 12) -> (junction 10)
    settings: description=无附加条件的迁移路径，执行次序1；沿本图当前连接推进。
  (junction 10) -> (junction 30)
    settings: description=无附加条件的迁移路径，执行次序1；沿本图当前连接推进。
  (junction 30) -> (junction 33) [order 1] : [Cnt/*计数器*/ < uint32/*三十二位无符号整数*/(Time_ms/*时间毫秒*//Ts_ms/*采样周期毫秒*/)]
    settings: description=本路径的判据/动作：[Cnt < uint32(Time_ms/Ts_ms)]。执行次序1；条件成立才执行本箭头动作。
  (junction 30) -> (junction 37) [order 2] : {ResetControl/*复位控制*/ = false/*假值*/;}
    settings: description=本路径的判据/动作：{ResetControl = false;}。执行次序2；条件成立才执行本箭头动作。
  (junction 33) -> (junction 36) : {ResetControl/*复位控制*/ = true/*真值*/;}
    settings: description=本路径的判据/动作：{ResetControl = true;}。执行次序1；条件成立才执行本箭头动作。
  (junction 36) -> (junction 37)
    settings: description=无附加条件的迁移路径，执行次序1；沿本图当前连接推进。
  (junction 37) -> (junction 55)
    settings: description=无附加条件的迁移路径，执行次序1；沿本图当前连接推进。
  (junction 55) -> (junction 43)
    settings: description=无附加条件的迁移路径，执行次序1；沿本图当前连接推进。
  (junction 43) -> (junction 71)
    settings: description=无附加条件的迁移路径，执行次序1；沿本图当前连接推进。
  data: Cnt local uint32 =0; ResetControl output boolean =0; Flag_ECUReset input boolean; Time_ms input single; Ts_ms parameter single

== stateflow chart turbo_controller/FPM/Subsystem/Hold_4000ms ==
  note: 闭环期间按约4 s间隔提出保存请求
      |
      | Flag_ClpControl为真时计数，为假时清零且不保存。当计数严格大于Time_ms/Ts_ms时，ECUReset_Sav
      | e给出真并清计数，随后重新开始下一轮。
      |
      | 当前Time_ms=4000、Ts_ms=20，比较门限200次，因采用“>”，事件会比恰好200拍多一个调用量级。
      | 它是周期性的保存触发，不是持续4 s都在发写命令。真正的多步FRAM写入由事务子系统完成。
  (default) -> (junction 26)
    settings: description=无附加条件的迁移路径，执行次序1；沿本图当前连接推进。
  (junction 26) -> (junction 3) [order 1] : [true/*真值*/ == Flag_ClpControl/*标志闭环控制*/]
    settings: description=本路径的判据/动作：[true == Flag_ClpControl]。执行次序1；条件成立才执行本箭头动作。
  (junction 3) -> (junction 5) [order 1] : [Cnt/*计数器*/ >= uint32/*三十二位无符号整数*/(10000)]
    settings: description=本路径的判据/动作：[Cnt >= uint32(10000)]。执行次序1；条件成立才执行本箭头动作。
  (junction 26) -> (junction 43) [order 2] : {Cnt/*计数器*/ = 0;
      | ECUReset_Save/*电子控制器复位保存*/ = false/*假值*/;}
    settings: description=本路径的判据/动作：{Cnt = 0; ECUReset_Save = false;}。执行次序2；条件成立才执行本箭头动作。
  (junction 3) -> (junction 10) [order 2] : {Cnt/*计数器*/++;}
    settings: description=本路径的判据/动作：{Cnt++;}。执行次序2；条件成立才执行本箭头动作。
  (junction 5) -> (junction 12) : {Cnt/*计数器*/ = 10000;}
    settings: description=本路径的判据/动作：{Cnt = 10000;}。执行次序1；条件成立才执行本箭头动作。
  (junction 12) -> (junction 10)
    settings: description=无附加条件的迁移路径，执行次序1；沿本图当前连接推进。
  (junction 10) -> (junction 30)
    settings: description=无附加条件的迁移路径，执行次序1；沿本图当前连接推进。
  (junction 30) -> (junction 33) [order 1] : [Cnt/*计数器*/ > uint32/*三十二位无符号整数*/(Time_ms/*时间毫秒*//Ts_ms/*采样周期毫秒*/)]
    settings: description=本路径的判据/动作：[Cnt > uint32(Time_ms/Ts_ms)]。执行次序1；条件成立才执行本箭头动作。
  (junction 30) -> (junction 37) [order 2] : {ECUReset_Save/*电子控制器复位保存*/ = false/*假值*/;}
    settings: description=本路径的判据/动作：{ECUReset_Save = false;}。执行次序2；条件成立才执行本箭头动作。
  (junction 33) -> (junction 36) : {ECUReset_Save/*电子控制器复位保存*/ = true/*真值*/;
      | Cnt/*计数器*/ = 0;}
    settings: description=本路径的判据/动作：{ECUReset_Save = true; Cnt = 0;}。执行次序1；条件成立才执行本箭头动作。
  (junction 36) -> (junction 37)
    settings: description=无附加条件的迁移路径，执行次序1；沿本图当前连接推进。
  (junction 37) -> (junction 55)
    settings: description=无附加条件的迁移路径，执行次序1；沿本图当前连接推进。
  (junction 55) -> (junction 43)
    settings: description=无附加条件的迁移路径，执行次序1；沿本图当前连接推进。
  (junction 43) -> (junction 71)
    settings: description=无附加条件的迁移路径，执行次序1；沿本图当前连接推进。
  data: Cnt local uint32 =0; ECUReset_Save output uint8 =0; Flag_ClpControl input uint8; Time_ms input single; Ts_ms parameter single

== stateflow chart turbo_controller/CLM/Manual/ManualAcc_Min_Control/Range ==
  note: 本实例把手动Data6限制在0～70，随后父级乘100变成泵给定0～7000。例如输入90先变70，再得到7000
      | 。
      |
      | 把一个数限制在允许范围内
      |
      | 输入包括待处理值、允许下限和允许上限。先比较是否越过上限，越过就输出上限；未超过上限时再检
      | 查下限，小于下限就输出下限；落在范围内则原样通过。恰好等于边界的值也保留。
      |
      | 计算式：输出 = min(max(输入，下限)，上限)。
      | 例如下限为0、上限为100时，输入120输出100，输入-5输出0，输入60输出60。这里不做平均、不计算
      | 变化速度，也不记住上一拍；它只防止当前数值越界。具体边界由父子系统连入，不能把此处的输出一
      | 律理解为百分比。
  (default) -> (junction 6)
    settings: description=无附加条件的迁移路径，执行次序1；沿本图当前连接推进。
  (junction 6) -> (junction 7) [order 1] : [In/*输入*/ <= Min/*下限*/]
    settings: description=本路径的判据/动作：[In <= Min]。执行次序1；条件成立才执行本箭头动作。
  (junction 6) -> (junction 29) [order 2] : {Out/*输出*/ = In/*输入*/;}
    settings: description=本路径的判据/动作：{Out = In;}。执行次序2；条件成立才执行本箭头动作。
  (junction 7) -> (junction 11) : {Out/*输出*/ = Min/*下限*/;}
    settings: description=本路径的判据/动作：{Out = Min;}。执行次序1；条件成立才执行本箭头动作。
  (junction 11) -> (junction 29)
    settings: description=无附加条件的迁移路径，执行次序1；沿本图当前连接推进。
  (junction 29) -> (junction 13)
    settings: description=无附加条件的迁移路径，执行次序1；沿本图当前连接推进。
  (junction 13) -> (junction 15) [order 1] : [Out/*输出*/ >= Max/*上限*/]
    settings: description=本路径的判据/动作：[Out >= Max]。执行次序1；条件成立才执行本箭头动作。
  (junction 13) -> (junction 20) [order 2]
    settings: description=无附加条件的迁移路径，执行次序2；沿本图当前连接推进。
  (junction 15) -> (junction 17) : {Out/*输出*/ = Max/*上限*/;}
    settings: description=本路径的判据/动作：{Out = Max;}。执行次序1；条件成立才执行本箭头动作。
  (junction 17) -> (junction 20)
    settings: description=无附加条件的迁移路径，执行次序1；沿本图当前连接推进。
  (junction 20) -> (junction 25)
    settings: description=无附加条件的迁移路径，执行次序1；沿本图当前连接推进。
  data: In input single; Max input single; Min input single; Out output single =0

== stateflow chart turbo_controller/MAM/Timmer_ms ==
  note: 确认越限是否持续达到指定时间
      |
      | 输入越限条件成立时累计次数；不成立时按图内复位分支清除本次确认。到Time_ms/Ts_ms对应的门限
      | 后，输出持续越限标志。
      |
      | 父级给定约2000 ms，Ts_ms=20 ms，相当于约100次连续调用。温度或转速只超过一拍后恢复，不会累
      | 计成连续2 s。该定时只用于告警确认，不改变测量值，也不对排温或转速再次滤波。
  (default) -> (junction 26)
    settings: description=无附加条件的迁移路径，执行次序1；沿本图当前连接推进。
  (junction 26) -> (junction 3) [order 1] : [true/*真值*/ == In/*输入*/]
    settings: description=本路径的判据/动作：[true == In]。执行次序1；条件成立才执行本箭头动作。
  (junction 3) -> (junction 5) [order 1] : [Cnt/*计数器*/ >= uint32/*三十二位无符号整数*/(100000)]
    settings: description=本路径的判据/动作：[Cnt >= uint32(100000)]。执行次序1；条件成立才执行本箭头动作。
  (junction 26) -> (junction 43) [order 2] : {Cnt/*计数器*/ = 0;Out/*输出*/ = false/*假值*/;}
    settings: description=本路径的判据/动作：{Cnt = 0;Out = false;}。执行次序2；条件成立才执行本箭头动作。
  (junction 3) -> (junction 10) [order 2] : {Cnt/*计数器*/++;}
    settings: description=本路径的判据/动作：{Cnt++;}。执行次序2；条件成立才执行本箭头动作。
  (junction 5) -> (junction 12) : {Cnt/*计数器*/ = 100000;}
    settings: description=本路径的判据/动作：{Cnt = 100000;}。执行次序1；条件成立才执行本箭头动作。
  (junction 12) -> (junction 10)
    settings: description=无附加条件的迁移路径，执行次序1；沿本图当前连接推进。
  (junction 10) -> (junction 30)
    settings: description=无附加条件的迁移路径，执行次序1；沿本图当前连接推进。
  (junction 30) -> (junction 33) [order 1] : [Cnt/*计数器*/ >uint32/*三十二位无符号整数*/(Time_ms/*时间毫秒*//Ts_ms/*采样周期毫秒*/)]
    settings: description=本路径的判据/动作：[Cnt >uint32(Time_ms/Ts_ms)]。执行次序1；条件成立才执行本箭头动作。
  (junction 30) -> (junction 37) [order 2] : {Out/*输出*/ = false/*假值*/;}
    settings: description=本路径的判据/动作：{Out = false;}。执行次序2；条件成立才执行本箭头动作。
  (junction 33) -> (junction 36) : {Out/*输出*/ = true/*真值*/;}
    settings: description=本路径的判据/动作：{Out = true;}。执行次序1；条件成立才执行本箭头动作。
  (junction 36) -> (junction 37)
    settings: description=无附加条件的迁移路径，执行次序1；沿本图当前连接推进。
  (junction 37) -> (junction 55)
    settings: description=无附加条件的迁移路径，执行次序1；沿本图当前连接推进。
  (junction 55) -> (junction 43)
    settings: description=无附加条件的迁移路径，执行次序1；沿本图当前连接推进。
  (junction 43) -> (junction 71)
    settings: description=无附加条件的迁移路径，执行次序1；沿本图当前连接推进。
  data: Cnt local uint32 =0; Out output boolean =0; In input boolean; Time_ms input single; Ts_ms parameter single

== stateflow chart turbo_controller/CLM/Manual/ManualAcc_Min_Control/手动加减/Hold_500ms ==
  note: 把一次触发延长成指定时长的操作窗口
      |
      | In为真，或上次尚在保持期间，就推进计数；否则把计数清零并令Out为假。在计数尚未达到Time_ms/T
      | s_ms时，Out为真并继续保持；达到门限后清计数、结束保持。
      |
      | 当前Ts_ms=20 ms，若Time_ms=500，门限为25次调用。输入只短暂来一次，也能在后续调用继续保持。
      | 这里输出的是窗口内外的布尔状态，不是“500 ms后才出现一次”的完成脉冲。计数还在1000处封顶，
      | 防止持续累加。
  (default) -> (junction 26)
    settings: description=无附加条件的迁移路径，执行次序1；沿本图当前连接推进。
  (junction 26) -> (junction 3) [order 1] : [true/*真值*/ == In/*输入*/ || Flag_Stay/*标志保持当前阶段*/]
    settings: description=本路径的判据/动作：[true == In || Flag_Stay]。执行次序1；条件成立才执行本箭头动作。
  (junction 3) -> (junction 5) [order 1] : [Cnt/*计数器*/ >= uint32/*三十二位无符号整数*/(1000)]
    settings: description=本路径的判据/动作：[Cnt >= uint32(1000)]。执行次序1；条件成立才执行本箭头动作。
  (junction 26) -> (junction 43) [order 2] : {Cnt/*计数器*/ = 0;Out/*输出*/ = false/*假值*/;}
    settings: description=本路径的判据/动作：{Cnt = 0;Out = false;}。执行次序2；条件成立才执行本箭头动作。
  (junction 3) -> (junction 10) [order 2] : {Cnt/*计数器*/++;}
    settings: description=本路径的判据/动作：{Cnt++;}。执行次序2；条件成立才执行本箭头动作。
  (junction 5) -> (junction 12) : {Cnt/*计数器*/ = 1000;}
    settings: description=本路径的判据/动作：{Cnt = 1000;}。执行次序1；条件成立才执行本箭头动作。
  (junction 12) -> (junction 10)
    settings: description=无附加条件的迁移路径，执行次序1；沿本图当前连接推进。
  (junction 10) -> (junction 30)
    settings: description=无附加条件的迁移路径，执行次序1；沿本图当前连接推进。
  (junction 30) -> (junction 33) [order 1] : [Cnt/*计数器*/ <uint32/*三十二位无符号整数*/(Time_ms/*时间毫秒*//Ts_ms/*采样周期毫秒*/)]
    settings: description=本路径的判据/动作：[Cnt <uint32(Time_ms/Ts_ms)]。执行次序1；条件成立才执行本箭头动作。
  (junction 30) -> (junction 37) [order 2] : {Cnt/*计数器*/ = 0;
      | Out/*输出*/ = false/*假值*/;
      | Flag_Stay/*标志保持当前阶段*/ = false/*假值*/;}
    settings: description=本路径的判据/动作：{Cnt = 0; Out = false; Flag_Stay = false;}。执行次序2；条件成立才执行本箭头动作。
  (junction 33) -> (junction 36) : {Out/*输出*/ = true/*真值*/;
      | Flag_Stay/*标志保持当前阶段*/ = true/*真值*/;}
    settings: description=本路径的判据/动作：{Out = true; Flag_Stay = true;}。执行次序1；条件成立才执行本箭头动作。
  (junction 36) -> (junction 37)
    settings: description=无附加条件的迁移路径，执行次序1；沿本图当前连接推进。
  (junction 37) -> (junction 55)
    settings: description=无附加条件的迁移路径，执行次序1；沿本图当前连接推进。
  (junction 55) -> (junction 43)
    settings: description=无附加条件的迁移路径，执行次序1；沿本图当前连接推进。
  (junction 43) -> (junction 71)
    settings: description=无附加条件的迁移路径，执行次序1；沿本图当前连接推进。
  data: Cnt local uint32 =0; Out output boolean =0; In input boolean; Time_ms input single; Ts_ms parameter single; Flag_Stay local boolean =0

== stateflow chart turbo_controller/CLM/Origin/Cool_Control ==
  note: 保留的停车冷却时序；当前请求端固定为0
      |
      | 本图用于收到冷却请求后按阶段控制起动电机、油泵及主油阀。Flag_Cool为假会撤销冷却过程、清总
      | 计数和完成标志；当前父系统把该输入接为常量0，因此这些主动冷却阶段目前不会投入。
      |
      | 若以后接入有效请求，图内有低转速检查和40、60等电机开通设定，并以30 s、40 s、50 s、70 s等计
      | 时点推进。供油支路按0.1×28/V_Power补偿供电变化；T4<110参与结束供油判断，120 s作为总流程退
      | 出限制。
      |
      | 时间比较采用毫秒/Time_ms换成调用次数，而不是每个计数代表1 s。V_Power来自父级选定信号，不能
      | 仅凭名称认定是ADC供电通道。此图保留算法，但实际是否运行由请求连接决定。
  (default) -> (junction 24)
    settings: description=无附加条件的迁移路径，执行次序1；沿本图当前连接推进。
  (junction 24) -> (junction 458) [order 1] : [Flag_Cool/*标志冷却*/  == true/*真值*/ && Flag_RunState/*标志运行状态*/~=4]
    settings: description=本路径的判据/动作：[Flag_Cool == true && Flag_RunState~=4]。执行次序1；条件成立才执行本箭头动作。
  (junction 24) -> (junction 964) [order 2]
    settings: description=无附加条件的迁移路径，执行次序2；沿本图当前连接推进。
  (junction 458) -> (junction 466) : {EarthStop/*地面停车*/ = true/*真值*/;}
    settings: description=本路径的判据/动作：{EarthStop = true;}。执行次序1；条件成立才执行本箭头动作。
  (junction 964) -> (junction 967) [order 1] : [Flag_Cool/*标志冷却*/  == false/*假值*/]
    settings: description=本路径的判据/动作：[Flag_Cool == false]。执行次序1；条件成立才执行本箭头动作。
  (junction 964) -> (junction 916) [order 2]
    settings: description=无附加条件的迁移路径，执行次序2；沿本图当前连接推进。
  (junction 967) -> (junction 969) : {EarthStop/*地面停车*/ = false/*假值*/;
      | CoolDoneFlag/*冷却完成标志*/ = false/*假值*/;
      | CNT_Global/*计数器全局*/=0;}
    settings: description=本路径的判据/动作：{EarthStop = false; CoolDoneFlag = false; CNT_Global=0;}。执行次序1；条件成立才执行本箭头动作。
  (junction 916) -> (junction 463)
    settings: description=无附加条件的迁移路径，执行次序1；沿本图当前连接推进。
  (junction 920) -> (junction 463)
    settings: description=无附加条件的迁移路径，执行次序1；沿本图当前连接推进。
  (junction 969) -> (junction 920)
    settings: description=无附加条件的迁移路径，执行次序1；沿本图当前连接推进。
  (junction 466) -> (junction 969)
    settings: description=无附加条件的迁移路径，执行次序1；沿本图当前连接推进。
  (junction 463) -> (junction 951)
    settings: description=无附加条件的迁移路径，执行次序1；沿本图当前连接推进。
  (junction 951) -> (junction 953) [order 1] : [CNT_Global/*计数器全局*/ >= (120000/Time_ms/*时间毫秒*/)]
    settings: description=本路径的判据/动作：[CNT_Global >= (120000/Time_ms)]。执行次序1；条件成立才执行本箭头动作。
  (junction 951) -> (junction 954) [order 2] : {CNT_Global/*计数器全局*/++;}
    settings: description=本路径的判据/动作：{CNT_Global++;}。执行次序2；条件成立才执行本箭头动作。
  (junction 953) -> (junction 959) : {CoolDoneFlag/*冷却完成标志*/ = true/*真值*/;
      | CNT_Global/*计数器全局*/ = 0;}
    settings: description=本路径的判据/动作：{CoolDoneFlag = true; CNT_Global = 0;}。执行次序1；条件成立才执行本箭头动作。
  (junction 959) -> (junction 954)
    settings: description=无附加条件的迁移路径，执行次序1；沿本图当前连接推进。
  (junction 954) -> (junction 830)
    settings: description=无附加条件的迁移路径，执行次序1；沿本图当前连接推进。
  (junction 830) -> (junction 829) [order 1] : [(EarthStop/*地面停车*/ == true/*真值*/) && (CoolDoneFlag/*冷却完成标志*/ == false/*假值*/)]
    settings: description=本路径的判据/动作：[(EarthStop == true) && (CoolDoneFlag == false)]。执行次序1；条件成立才执行本箭头动作。
  (junction 829) -> (junction 833) [order 1] : [Nc/*发动机反馈转速（转每分）*/ < 2000]
    settings: description=本路径的判据/动作：[Nc < 2000]。执行次序1；条件成立才执行本箭头动作。
  (junction 830) -> (junction 907) [order 2] : {Accelerator/*油门／油泵给定控制量*/ = single/*单精度浮点*/(0);
      | EValve_Open/*主油阀开通计数（每计数2毫秒）*/ = uint16/*十六位无符号整数*/(0);
      | Motor_Open/*起动电机开通计数*/ = uint16/*十六位无符号整数*/(0);
      | EValve_Enable/*主油阀驱动使能*/ = uint8/*八位无符号整数*/(0);
      | Motor_Enable/*起动电机使能*/ = uint8/*八位无符号整数*/(0);}
    settings: description=本路径的判据/动作：{Accelerator = single(0); EValve_Open = uint16(0); Motor_Open = uint16(0); EValve_Enable = uint8(0); Motor_Enable = uint8(0);}。执行次序2；条件成立才执行本箭头动作。
  (junction 829) -> (junction 839) [order 2] : {Accelerator/*油门／油泵给定控制量*/ = single/*单精度浮点*/(0);
      | EValve_Open/*主油阀开通计数（每计数2毫秒）*/ = uint16/*十六位无符号整数*/(0);
      | Motor_Open/*起动电机开通计数*/ = uint16/*十六位无符号整数*/(0);
      | EValve_Enable/*主油阀驱动使能*/ = uint8/*八位无符号整数*/(0);
      | Motor_Enable/*起动电机使能*/ = uint8/*八位无符号整数*/(0);}
    settings: description=本路径的判据/动作：{Accelerator = single(0); EValve_Open = uint16(0); Motor_Open = uint16(0); EValve_Enable = uint8(0); Motor_Enable = uint8(0);}。执行次序2；条件成立才执行本箭头动作。
  (junction 833) -> (junction 837) : {Motor_Open/*起动电机开通计数*/ = uint16/*十六位无符号整数*/(40);
      | Motor_Enable/*起动电机使能*/ = uint8/*八位无符号整数*/(1);}
    settings: description=本路径的判据/动作：{Motor_Open = uint16(40); Motor_Enable = uint8(1);}。执行次序1；条件成立才执行本箭头动作。
  (junction 837) -> (junction 839)
    settings: description=无附加条件的迁移路径，执行次序1；沿本图当前连接推进。
  (junction 839) -> (junction 855)
    settings: description=无附加条件的迁移路径，执行次序1；沿本图当前连接推进。
  (junction 855) -> (junction 857) [order 1] : [CNT_EarthCoolTime/*计数器地面冷却时间*/ >= (30000/Time_ms/*时间毫秒*/) && Flag_RunState/*标志运行状态*/~=15]
    settings: description=本路径的判据/动作：[CNT_EarthCoolTime >= (30000/Time_ms) && Flag_RunState~=15]。执行次序1；条件成立才执行本箭头动作。
  (junction 855) -> (junction 861) [order 2]
    settings: description=无附加条件的迁移路径，执行次序2；沿本图当前连接推进。
  (junction 857) -> (junction 859) : {Accelerator/*油门／油泵给定控制量*/ = single/*单精度浮点*/(0.1*28/V_Power/*电压或控制量变量电源*/);
      | EValve_Open/*主油阀开通计数（每计数2毫秒）*/ = uint16/*十六位无符号整数*/(30);
      | Motor_Open/*起动电机开通计数*/ = uint16/*十六位无符号整数*/(60);
      | EValve_Enable/*主油阀驱动使能*/ = uint8/*八位无符号整数*/(1);
      | Motor_Enable/*起动电机使能*/ = uint8/*八位无符号整数*/(1);}
    settings: description=本路径的判据/动作：{Accelerator = single(0.1*28/V_Power); EValve_Open = uint16(30); Motor_Open = uint16(60); EValve_Enable = uint8(1); Motor_Enable = uint8(1);}。执行次序1；条件成立才执行本箭头动作。
  (junction 859) -> (junction 861)
    settings: description=无附加条件的迁移路径，执行次序1；沿本图当前连接推进。
  (junction 861) -> (junction 864)
    settings: description=无附加条件的迁移路径，执行次序1；沿本图当前连接推进。
  (junction 864) -> (junction 866) [order 1] : [CNT_EarthCoolTime/*计数器地面冷却时间*/ >= (40000/Time_ms/*时间毫秒*/)]
    settings: description=本路径的判据/动作：[CNT_EarthCoolTime >= (40000/Time_ms)]。执行次序1；条件成立才执行本箭头动作。
  (junction 866) -> (junction 868) [order 1] : [(T4_Filter/*滤波排温*/ < 110) ||...
      | (CNT_EarthCoolTime/*计数器地面冷却时间*/ >= (50000/Time_ms/*时间毫秒*/))]
    settings: description=本路径的判据/动作：[(T4_Filter < 110) ||... (CNT_EarthCoolTime >= (50000/Time_ms))]。执行次序1；条件成立才执行本箭头动作。
  (junction 864) -> (junction 875) [order 2]
    settings: description=无附加条件的迁移路径，执行次序2；沿本图当前连接推进。
  (junction 866) -> (junction 872) [order 2] : {Accelerator/*油门／油泵给定控制量*/ = single/*单精度浮点*/(0);}
    settings: description=本路径的判据/动作：{Accelerator = single(0);}。执行次序2；条件成立才执行本箭头动作。
  (junction 868) -> (junction 870) : {Accelerator/*油门／油泵给定控制量*/ = single/*单精度浮点*/(0);
      | EValve_Open/*主油阀开通计数（每计数2毫秒）*/ = uint16/*十六位无符号整数*/(0);
      | EValve_Enable/*主油阀驱动使能*/ = uint8/*八位无符号整数*/(0);
      | Motor_Open/*起动电机开通计数*/ = uint16/*十六位无符号整数*/(0);}
    settings: description=本路径的判据/动作：{Accelerator = single(0); EValve_Open = uint16(0); EValve_Enable = uint8(0); Motor_Open = uint16(0);}。执行次序1；条件成立才执行本箭头动作。
  (junction 872) -> (junction 875)
    settings: description=无附加条件的迁移路径，执行次序1；沿本图当前连接推进。
  (junction 870) -> (junction 872)
    settings: description=无附加条件的迁移路径，执行次序1；沿本图当前连接推进。
  (junction 875) -> (junction 878)
    settings: description=无附加条件的迁移路径，执行次序1；沿本图当前连接推进。
  (junction 878) -> (junction 880) [order 1] : [CNT_EarthCoolTime/*计数器地面冷却时间*/ >= (70000/Time_ms/*时间毫秒*/)]
    settings: description=本路径的判据/动作：[CNT_EarthCoolTime >= (70000/Time_ms)]。执行次序1；条件成立才执行本箭头动作。
  (junction 878) -> (junction 884) [order 2] : {CNT_EarthCoolTime/*计数器地面冷却时间*/++;}
    settings: description=本路径的判据/动作：{CNT_EarthCoolTime++;}。执行次序2；条件成立才执行本箭头动作。
  (junction 880) -> (junction 771) : {Accelerator/*油门／油泵给定控制量*/ = single/*单精度浮点*/(0);
      | EValve_Open/*主油阀开通计数（每计数2毫秒）*/ = uint16/*十六位无符号整数*/(0);
      | Motor_Open/*起动电机开通计数*/ = uint16/*十六位无符号整数*/(0);
      | EValve_Enable/*主油阀驱动使能*/ = uint8/*八位无符号整数*/(0);
      | Motor_Enable/*起动电机使能*/ = uint8/*八位无符号整数*/(0);
      | CNT_EarthCoolTime/*计数器地面冷却时间*/ = 0;
      | CoolDoneFlag/*冷却完成标志*/ = true/*真值*/;}
    settings: description=本路径的判据/动作：{Accelerator = single(0); EValve_Open = uint16(0); Motor_Open = uint16(0); EValve_Enable = uint8(0); Motor_Enable = uint8(0); CNT_EarthCoolTime = 0; CoolDoneFlag = true;}。执行次序1；条件成立才执行本箭头动作。
  (junction 884) -> (junction 907)
    settings: description=无附加条件的迁移路径，执行次序1；沿本图当前连接推进。
  (junction 771) -> (junction 884)
    settings: description=无附加条件的迁移路径，执行次序1；沿本图当前连接推进。
  (junction 907) -> (junction 910)
    settings: description=无附加条件的迁移路径，执行次序1；沿本图当前连接推进。
  data: Time_ms input single; Accelerator output single =0; Nc input single; T4_Filter input single; Flag_Cool input boolean; V_Power input single; EValve_Open output uint16 =0; Motor_Open output uint16 =0; EValve_Enable output uint8 =0; Motor_Enable output uint8 =0; EarthStop local boolean =0; CNT_EarthCoolTime local uint32 =0; CNT_Global local uint32 =0; CoolDoneFlag local boolean =0; Flag_RunState input uint8

== stateflow chart turbo_controller/CLM/Start/HoldFirst/Hold ==
  note: 识别本次执行的第一次调用
      |
      | 内部保持一个首次标志。第一次进入时给出用于初始化的标志，之后把内部状态切换为已经执行，使后
      | 续调用采用保持或正常处理路径。
      |
      | 本图自身不存储温度、油压或参数数组。需要保留的具体数值在父系统的开关与延迟中保存；本图只告
      | 诉父系统何时取初值。它也不是每拍都产生一次上升沿。重新初始化模型时会重新开始这一首次判断。
  (default) -> (junction 26)
    settings: description=无附加条件的迁移路径，执行次序1；沿本图当前连接推进。
  (junction 26) -> (junction 3) [order 1] : [true/*真值*/ == Flag_First/*标志首次*/]
    settings: description=本路径的判据/动作：[true == Flag_First]。执行次序1；条件成立才执行本箭头动作。
  (junction 26) -> (junction 43) [order 2] : {Out/*输出*/ = true/*真值*/;
      | Flag_First/*标志首次*/ = true/*真值*/;}
    settings: description=本路径的判据/动作：{Out = true; Flag_First = true;}。执行次序2；条件成立才执行本箭头动作。
  (junction 3) -> (junction 55) : {Out/*输出*/ = false/*假值*/;}
    settings: description=本路径的判据/动作：{Out = false;}。执行次序1；条件成立才执行本箭头动作。
  (junction 55) -> (junction 43)
    settings: description=无附加条件的迁移路径，执行次序1；沿本图当前连接推进。
  (junction 43) -> (junction 71)
    settings: description=无附加条件的迁移路径，执行次序1；沿本图当前连接推进。
  data: Out output boolean =0; Flag_First local boolean =0

== stateflow chart turbo_controller/CLM/Manual/ManualEValve_Control/Range ==
  note: 本实例限制主油阀开通计数0～30。周期固定30，换算值15表示半周期开通；板级2 ms节拍下对应开30
      | ms、关30 ms。
      |
      | 把一个数限制在允许范围内
      |
      | 输入包括待处理值、允许下限和允许上限。先比较是否越过上限，越过就输出上限；未超过上限时再检
      | 查下限，小于下限就输出下限；落在范围内则原样通过。恰好等于边界的值也保留。
      |
      | 计算式：输出 = min(max(输入，下限)，上限)。
      | 例如下限为0、上限为100时，输入120输出100，输入-5输出0，输入60输出60。这里不做平均、不计算
      | 变化速度，也不记住上一拍；它只防止当前数值越界。具体边界由父子系统连入，不能把此处的输出一
      | 律理解为百分比。
  (default) -> (junction 6)
    settings: description=无附加条件的迁移路径，执行次序1；沿本图当前连接推进。
  (junction 6) -> (junction 7) [order 1] : [In/*输入*/ <= Min/*下限*/]
    settings: description=本路径的判据/动作：[In <= Min]。执行次序1；条件成立才执行本箭头动作。
  (junction 6) -> (junction 29) [order 2] : {Out/*输出*/ = In/*输入*/;}
    settings: description=本路径的判据/动作：{Out = In;}。执行次序2；条件成立才执行本箭头动作。
  (junction 7) -> (junction 11) : {Out/*输出*/ = Min/*下限*/;}
    settings: description=本路径的判据/动作：{Out = Min;}。执行次序1；条件成立才执行本箭头动作。
  (junction 11) -> (junction 29)
    settings: description=无附加条件的迁移路径，执行次序1；沿本图当前连接推进。
  (junction 29) -> (junction 13)
    settings: description=无附加条件的迁移路径，执行次序1；沿本图当前连接推进。
  (junction 13) -> (junction 15) [order 1] : [Out/*输出*/ >= Max/*上限*/]
    settings: description=本路径的判据/动作：[Out >= Max]。执行次序1；条件成立才执行本箭头动作。
  (junction 13) -> (junction 20) [order 2]
    settings: description=无附加条件的迁移路径，执行次序2；沿本图当前连接推进。
  (junction 15) -> (junction 17) : {Out/*输出*/ = Max/*上限*/;}
    settings: description=本路径的判据/动作：{Out = Max;}。执行次序1；条件成立才执行本箭头动作。
  (junction 17) -> (junction 20)
    settings: description=无附加条件的迁移路径，执行次序1；沿本图当前连接推进。
  (junction 20) -> (junction 25)
    settings: description=无附加条件的迁移路径，执行次序1；沿本图当前连接推进。
  data: In input single; Max input single; Min input single; Out output single =0

== stateflow chart turbo_controller/CLM/Manual/Eblast_Control/Range ==
  note: 本实例限制副油阀开通计数0～30，对应固定周期30。计算值45限制为30，最多整个周期都开，不会出
      | 现开通时间大于周期。
      |
      | 把一个数限制在允许范围内
      |
      | 输入包括待处理值、允许下限和允许上限。先比较是否越过上限，越过就输出上限；未超过上限时再检
      | 查下限，小于下限就输出下限；落在范围内则原样通过。恰好等于边界的值也保留。
      |
      | 计算式：输出 = min(max(输入，下限)，上限)。
      | 例如下限为0、上限为100时，输入120输出100，输入-5输出0，输入60输出60。这里不做平均、不计算
      | 变化速度，也不记住上一拍；它只防止当前数值越界。具体边界由父子系统连入，不能把此处的输出一
      | 律理解为百分比。
  (default) -> (junction 6)
    settings: description=无附加条件的迁移路径，执行次序1；沿本图当前连接推进。
  (junction 6) -> (junction 7) [order 1] : [In/*输入*/ <= Min/*下限*/]
    settings: description=本路径的判据/动作：[In <= Min]。执行次序1；条件成立才执行本箭头动作。
  (junction 6) -> (junction 29) [order 2] : {Out/*输出*/ = In/*输入*/;}
    settings: description=本路径的判据/动作：{Out = In;}。执行次序2；条件成立才执行本箭头动作。
  (junction 7) -> (junction 11) : {Out/*输出*/ = Min/*下限*/;}
    settings: description=本路径的判据/动作：{Out = Min;}。执行次序1；条件成立才执行本箭头动作。
  (junction 11) -> (junction 29)
    settings: description=无附加条件的迁移路径，执行次序1；沿本图当前连接推进。
  (junction 29) -> (junction 13)
    settings: description=无附加条件的迁移路径，执行次序1；沿本图当前连接推进。
  (junction 13) -> (junction 15) [order 1] : [Out/*输出*/ >= Max/*上限*/]
    settings: description=本路径的判据/动作：[Out >= Max]。执行次序1；条件成立才执行本箭头动作。
  (junction 13) -> (junction 20) [order 2]
    settings: description=无附加条件的迁移路径，执行次序2；沿本图当前连接推进。
  (junction 15) -> (junction 17) : {Out/*输出*/ = Max/*上限*/;}
    settings: description=本路径的判据/动作：{Out = Max;}。执行次序1；条件成立才执行本箭头动作。
  (junction 17) -> (junction 20)
    settings: description=无附加条件的迁移路径，执行次序1；沿本图当前连接推进。
  (junction 20) -> (junction 25)
    settings: description=无附加条件的迁移路径，执行次序1；沿本图当前连接推进。
  data: In input single; Max input single; Min input single; Out output single =0

== stateflow chart turbo_controller/CLM/Manual/Motor_Control/Range ==
  note: 本实例限制手动电机开通计数0～100，周期100。设定120只输出100，不会超过满周期；使能还由父级
      | 单独判断。
      |
      | 把一个数限制在允许范围内
      |
      | 输入包括待处理值、允许下限和允许上限。先比较是否越过上限，越过就输出上限；未超过上限时再检
      | 查下限，小于下限就输出下限；落在范围内则原样通过。恰好等于边界的值也保留。
      |
      | 计算式：输出 = min(max(输入，下限)，上限)。
      | 例如下限为0、上限为100时，输入120输出100，输入-5输出0，输入60输出60。这里不做平均、不计算
      | 变化速度，也不记住上一拍；它只防止当前数值越界。具体边界由父子系统连入，不能把此处的输出一
      | 律理解为百分比。
  (default) -> (junction 6)
    settings: description=无附加条件的迁移路径，执行次序1；沿本图当前连接推进。
  (junction 6) -> (junction 7) [order 1] : [In/*输入*/ <= Min/*下限*/]
    settings: description=本路径的判据/动作：[In <= Min]。执行次序1；条件成立才执行本箭头动作。
  (junction 6) -> (junction 29) [order 2] : {Out/*输出*/ = In/*输入*/;}
    settings: description=本路径的判据/动作：{Out = In;}。执行次序2；条件成立才执行本箭头动作。
  (junction 7) -> (junction 11) : {Out/*输出*/ = Min/*下限*/;}
    settings: description=本路径的判据/动作：{Out = Min;}。执行次序1；条件成立才执行本箭头动作。
  (junction 11) -> (junction 29)
    settings: description=无附加条件的迁移路径，执行次序1；沿本图当前连接推进。
  (junction 29) -> (junction 13)
    settings: description=无附加条件的迁移路径，执行次序1；沿本图当前连接推进。
  (junction 13) -> (junction 15) [order 1] : [Out/*输出*/ >= Max/*上限*/]
    settings: description=本路径的判据/动作：[Out >= Max]。执行次序1；条件成立才执行本箭头动作。
  (junction 13) -> (junction 20) [order 2]
    settings: description=无附加条件的迁移路径，执行次序2；沿本图当前连接推进。
  (junction 15) -> (junction 17) : {Out/*输出*/ = Max/*上限*/;}
    settings: description=本路径的判据/动作：{Out = Max;}。执行次序1；条件成立才执行本箭头动作。
  (junction 17) -> (junction 20)
    settings: description=无附加条件的迁移路径，执行次序1；沿本图当前连接推进。
  (junction 20) -> (junction 25)
    settings: description=无附加条件的迁移路径，执行次序1；沿本图当前连接推进。
  data: In input single; Max input single; Min input single; Out output single =0

== stateflow chart turbo_controller/FPM/Up_Hold ==
  note: 把复位请求锁住，避免一拍命令丢失
      |
      | 输入In一旦为真，就把Out置为真。图内没有输入变假就清Out的对应动作，因此它是请求锁存，而不是
      | 简单复制输入，也不是单拍脉冲。
      |
      | 后续模式与事务逻辑可以在命令消失后继续看到请求。锁存状态在模型或图初始化时重置；此图不等待
      | SPI完成，也不表示硬件复位已经执行。
  (default) -> (junction 26)
    settings: description=无附加条件的迁移路径，执行次序1；沿本图当前连接推进。
  (junction 26) -> (junction 3) [order 1] : [true/*真值*/ == In/*输入*/]
    settings: description=本路径的判据/动作：[true == In]。执行次序1；条件成立才执行本箭头动作。
  (junction 26) -> (junction 43) [order 2]
    settings: description=无附加条件的迁移路径，执行次序2；沿本图当前连接推进。
  (junction 3) -> (junction 55) : {Out/*输出*/ = true/*真值*/;}
    settings: description=本路径的判据/动作：{Out = true;}。执行次序1；条件成立才执行本箭头动作。
  (junction 55) -> (junction 43)
    settings: description=无附加条件的迁移路径，执行次序1；沿本图当前连接推进。
  (junction 43) -> (junction 71)
    settings: description=无附加条件的迁移路径，执行次序1；沿本图当前连接推进。
  data: Out output boolean =0; In input boolean =0
